simulink model "FS_PWT_Full_Assembly"  (R2025b)
settings: Solver=ode1  StartTime=0.0  StopTime=17  FixedStep=0.05*1/f_sw  RelTol=1e-3
values from neighbouring files (symbols this model uses):
  f_sw = 10000    [Example_parameters.m]
  G_off = 1e-6    (= 1e-06)    [Example_parameters.m]
  J_m = 2.74e-4    (= 0.000274)    [Example_parameters.m]
  k_T = 0.208    [Example_parameters.m]
  n_max = 20000    [Example_parameters.m]
  nm_ref = n_max    (= 20000)    [Example_parameters.m]
  p = 5    [Example_parameters.m]
  R_ds = 0.01    [Example_parameters.m]
  t0 = 0.2    [Example_parameters.m]
  T1 = 0.9*T_max    (= 18)    [Example_parameters.m]
  t1 = t0+5    (= 5.2)    [Example_parameters.m]
  T2 = -T_rated    (= -9.8)    [Example_parameters.m]
  t2 = t1+10    (= 15.2)    [Example_parameters.m]
  Torque_set_matrix = [379.08 379.13 379.18 379.23 379.28 379.33 379.38 379.43 379.48 379.53 379.58 379.63 ... (678 elements, 339x2)]    [Example_torque_reference.mat]
  V_dc = 600    [Example_parameters.m]
  V_th = 2    [Example_parameters.m]
libraries: nesl_utility x15, ee_lib x11, fl_lib x9, eeTransforms x3, simulink x1
settings Model: SimulationMode=accelerator  Creator=giuli  LastModifiedBy=test

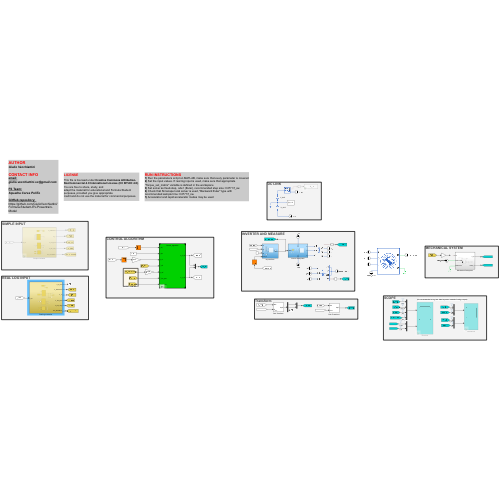
[thumbnail: Simulink's stored preview of the top-level diagram]
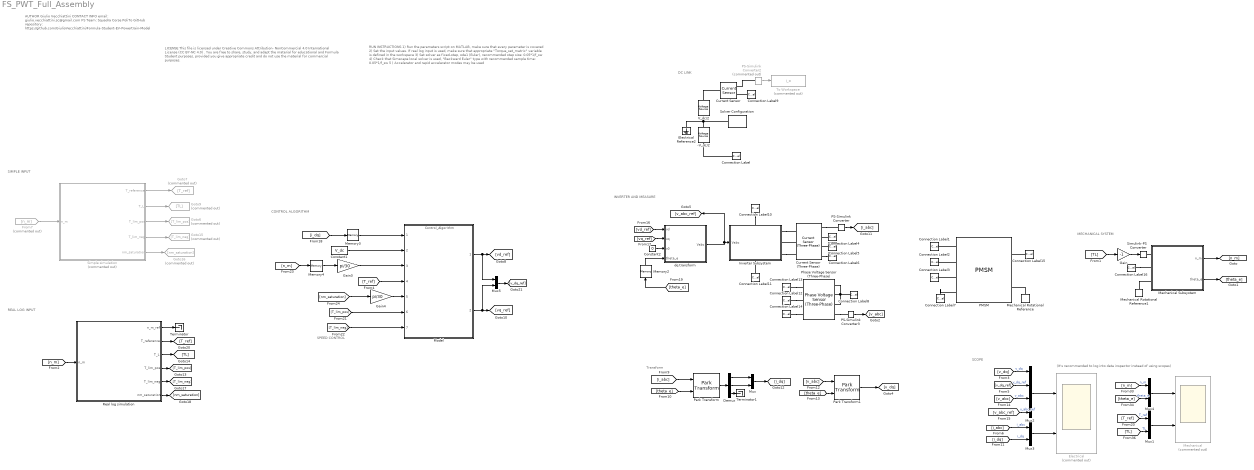
== system FS_PWT_Full_Assembly ==
  note: LICENSE
      |
      | This file is licensed under Creative Commons Attribution-
      | NonCommercial 4.0 International License (CC BY-NC 4.0) . You are free to share, study, and
      | adapt the material for educational and Formula Student purposes, provided you give appropriate
      | credit and do not use the material for commercial purposes.
  note: REAL LOG INPUT
  note: SCOPE
  note: INVERTER AND MEASURE
  note: RUN INSTRUCTIONS
      | 1) Run the parameters script on MATLAB, make sure that every parameter is covered
      | 2) Set the input values. If real log input is used, make sure that appropriate "Torque_set_matrix" variable is defined in the workspace
      | 3) Set solver as fixed-step, ode1 (Euler), recommended step size: 0.05*1/f_sw
      | 4) Check that Simscape local solver is used, "Backward Euler" type with recommended sample time: 0.05*1/f_sw
      | 5 ) Accelerator and rapid accelerator modes may be used
  note: SIMPLE INPUT
  note: DC LINK
  note: Transform
  note: SPEED CONTROL
  note: MECHANICAL SYSTEM
  note: CONTROL ALGORITHM
  note: AUTHOR
      | Giulio Vecchiattini
      |
      | CONTACT INFO
      | email: giulio.vecchiattini.sc@gmail.com
      |
      | FS Team:
      | Squadra Corse PoliTo
      |
      | GitHub repository:
      | https://github.com/GiulioVecchiattini/Formula-Student-EV-Powertrain-Model
  note: (It's recommended to log into data inspector instead of using scopes)
  -V_dc/2 : ee_lib/Sources/Voltage Source  dc_voltage=V_dc/2 V  ac_voltage=0 V  ac_shift=0 rad  ac_frequency=0 Hz  noise_mode=ee.enum.sources.noise.Disabled  PSD=0 V^2/Hz  sample_time=1e-3 s  repeatability=ee.enum.sources.repeatability.NotRepeatable  user_seed=0  auto_seed=2715962282  i_specify=off  i_priority=None  i=0 A  i_nominal_specify=off  i_nominal_value=1  i_nominal_unit=A  v_specify=off  v_priority=None  v=0 V  v_nominal_specify=off  v_nominal_value=1  v_nominal_unit=V
  Connection Label : ConnectionLabel  Label=Neg
  Connection Label1 : ConnectionLabel  Label=v_a
  Connection Label10 : ConnectionLabel  Label=V_dc
  Connection Label11 : ConnectionLabel  Label=Neg
  Connection Label12 : ConnectionLabel  Label=v_b
  Connection Label13 : ConnectionLabel  Label=v_c
  Connection Label14 : ConnectionLabel  Label=v_a
  Connection Label15 : ConnectionLabel  Label=Rotor_shaft
  Connection Label16 : ConnectionLabel  Label=Rotor_shaft
  Connection Label2 : ConnectionLabel  Label=v_b
  Connection Label3 : ConnectionLabel  Label=v_c
  Connection Label4 : ConnectionLabel  Label=v_a
  Connection Label5 : ConnectionLabel  Label=v_b
  Connection Label6 : ConnectionLabel  Label=v_c
  Connection Label7 : ConnectionLabel  Label=motor_ground
  Connection Label8 : ConnectionLabel  Label=motor_ground
  Connection Label9 : ConnectionLabel  Label=V_dc
  Constant1 : Constant  Value=V_dc
  Constant2 : Constant  Value=0
  Current Sensor : fl_lib/Electrical/Electrical Sensors/Current Sensor
  Current Sensor (Three-Phase) : ee_lib/Sensors & Transducers/Current Sensor (Three-Phase)
      settings: InternalSimscapePortConfiguration="{\"Bottom\":[],\"Left\":[{\"id\":\"a1\",\"label\":\"a1\",\"type\":\"foundation.electrical.electrical\"},{\"id\":\"b1\",\"label\":\"b1\",\"type\":\"foundation.electrical.electrical\"},{\"id\":\"c1\",\"label\":\"c1\",\"type\":\"foundation.electrical.electrical\"}],\"Right\":[{\"id\":\"I_output\",\"label\":\"I\",\"type\":\"output\"},{\"id\":\"a2\",\"label\":\"a2\",\"type\":\"foundation.electrical.electrical\"},{\"id\":\"b2\",\"label\":\"b2\",\"type\":\"foundation.electrical.electrical\"},{\"id\":\"c2\",\"label\":\"c2\",\"type\":\"foundation.electrical.electrical\"}],\"Top\":[]}"
  Demux : Demux  Outputs=3
  Electrical : Scope  Commented=on  NumInputPorts=2
      settings: ActiveDisplayYMinimum=-254.85497098950052  ActiveDisplayYMaximum=280.09054138194477
  Electrical Reference2 : fl_lib/Electrical/Electrical Elements/Electrical Reference
  From7 : From  Commented=on  GotoTag=n_m
  Gain : Gain  Gain=-1
  Gain3 : Gain  Gain=pi/30
  Gain4 : Gain  Gain=pi/30
  Goto15 : Goto  Commented=on  GotoTag=T_lim_neg
  Goto16 : Goto  Commented=on  GotoTag=nm_saturation
  Goto6 : Goto  Commented=on  GotoTag=T_lim_pos
  Goto7 : Goto  Commented=on  GotoTag=T_ref
  Goto9 : Goto  Commented=on  GotoTag=TL
  Inverter Subsystem : Subsystem
      settings: PortSchema="{\"entries\":[{\"content\":{\"sides\":[{\"content\":{\"connectorIds\":[\"In1\"]},\"type\":\"ConnectorPlacement.EquallySpacedRectSide\",\"uuid\":\"d192f5af-ddff-4fda-a54c-c11e3916a7bb\"},{\"content\":{\"connectorIds\":[\"RConn1\",\"RConn2\",\"RConn3\"],\"side\":\"RIGHT\"},\"type\":\"ConnectorPlacement.EquallySpacedRectSide\",\"uuid\":\"2c430e4a-8be9-4c5f-98fc-1673ba6cdbf8\"},{\"content\":{\"connectorIds\":[\"LConn1\"],\"side\":\"TOP\"},\"type\":\"ConnectorPlacement.EquallySpacedRectSide\",\"uuid\":\"e498738c-bc20-41e6-88d8-a49171ce1bf1\"},{\"content\":{\"connectorIds\":[\"RConn4\"],\"side\":\"BOTTOM\"},\"type\":\"ConnectorPlacement.EquallySpacedRectSide\",\"uuid\":\"b8f4106f-31ca-4add-9d4b-ac081118ee10\"}]},\"type\":\"ConnectorPlacement.EquallySpacedConnector\",\"uuid\":\"9fb2183f-2e1f-4b7b-94f3-85e82ac3160c\"}],\"packageUris\":[\"http://schema.mathworks.com/mf0/Connector/R2020b\"],\"version\":\"1.0\"}"
  Mechanical : Scope  Commented=on  NumInputPorts=2
      settings: ActiveDisplayYMinimum=-2480.3611684593266  ActiveDisplayYMaximum=22322.963570599019  DataLoggingVariableName=ScopeData5
  Mechanical Rotational Reference : fl_lib/Mechanical/Rotational Elements/Mechanical Rotational Reference
  Mechanical Rotational Reference1 : fl_lib/Mechanical/Rotational Elements/Mechanical Rotational Reference
  Mechanical Subsystem : Subsystem
  Memory2 : Memory
  Memory3 : Memory
  Memory4 : Memory
  Model : ModelReference  ModelNameDialog=Control_Algorithm.slxp  UsingDefaultArgumentValue=0,0,0,0,0,0,0,0,0,0,0,0,0,0,0,0,0,0,0  ModelReferenceVersion=1.7  CopyOfModelProtected=on  Torque_control=0  T_max=T_max  V_dc_max=V_dc_max  V_max=V_max  k_T=k_T  I_max=I_max  Kp_d=Kp_d  Ki_d=Ki_d  Kp_q=Kp_q  Ki_q=Ki_q  Kp_n=Kp_n  Ki_n=Ki_n  Kd_n=Kd_n  Kp_v=Kp_v  Ki_v=Ki_v  n_lim_brake=0.02*n_max  n_min_brake=0.01*n_max  n_max=n_max*1.02  n_lim=0.95*n_max
  Mux{,1,3..5} (5 alike) : Mux  Inputs=2
  Mux2 : Mux
  PMSM : ee_lib/Electromechanical/Permanent Magnet/PMSM  port_option=ee.enum.threePhasePort.expanded  winding_type=ee.enum.electromech.statorconfiguration.wye  machine_param=ee.enum.pmsm.parameterization.constant  nPolePairs=p  pmflux_param=ee.enum.pmflux.fluxlinkage  pm_flux_linkage=Fm Wb  torque_constant=k_T*0.8 N*m/A  back_emf_constant=0.18 V*s/rad  stator_param=ee.enum.statorparam.LdLqL0  Ld=Ld H  Lq=Lq H  idVec=[-200, 0, 200] A  iqVec=[-200, 0, 200] A  LdMatrix=0.0002 * ones(3, 3) H  LqMatrix=0.0002 * ones(3, 3) H  PmMatrix=0.1 * ones(3, 3) Wb  ktMatrix=0.18 * ones(3, 3) N*m/A  keMatrix=0.18 * ones(3, 3) V*s/rad  L0=L0 H  Ls=0.0002 H  Lm=-0.00002 H  Ms=0.00002 H  Rs=R_s Ohm  zero_sequence=ee.enum.park.zerosequence.include  axes_param=ee.enum.rotorangle.daxis  loss_param=ee.enum.ironloss.none  losses_oc=[0, 0, 0] W  losses_sc=[0, 0, 0] W  f_losses=60 Hz  Isc_losses=95 A  J=J_m kg*m^2  lam=B_m N*m*s/rad  i_d_specify=off  i_d_priority=None  i_d=0 A  i_d_nominal_specify=off  i_d_nominal_value=1  i_d_nominal_unit=A  i_q_specify=off  i_q_priority=None  i_q=0 A  i_q_nominal_specify=off  i_q_nominal_value=1  i_q_nominal_unit=A  torque_specify=off  torque_priority=None  torque=0 N*m  torque_nominal_specify=off  torque_nominal_value=1  torque_nominal_unit=N*m  angular_velocity_specify=off  angular_velocity_priority=High  angular_velocity=0 rpm  angular_velocity_nominal_specify=off  angular_velocity_nominal_value=1  angular_velocity_nominal_unit=rpm  angular_position_specify=off  angular_position_priority=High  angular_position=0 deg  angular_position_nominal_specify=off  angular_position_nominal_value=1  angular_position_nominal_unit=deg  alpha=3.93e-3 1/K  alpha_flux=-0.001 1/K  Tmeas=298.15 K  stator_thermal_mass=100 J/K  rotor_thermal_mass=200 J/K  Rm_percent_rotor=90  Rd_percent_rotor=30  temperatureA_specify=off  temperatureA_priority=High  temperatureA=25 degC  temperatureA_nominal_specify=off  temperatureA_nominal_value=1  temperatureA_nominal_unit=degC  temperatureB_specify=off  temperatureB_priority=High  temperatureB=25 degC  temperatureB_nominal_specify=off  temperatureB_nominal_value=1  temperatureB_nominal_unit=degC  temperatureC_specify=off  temperatureC_priority=High  temperatureC=25 degC  temperatureC_nominal_specify=off  temperatureC_nominal_value=1  temperatureC_nominal_unit=degC  temperatureR_specify=off  temperatureR_priority=High  temperatureR=25 degC  temperatureR_nominal_specify=off  temperatureR_nominal_value=1  temperatureR_nominal_unit=degC
      settings: InternalSimscapePortConfiguration="{\"Bottom\":[],\"Left\":[{\"id\":\"a\",\"label\":\"a\",\"type\":\"foundation.electrical.electrical\"},{\"id\":\"b\",\"label\":\"b\",\"type\":\"foundation.electrical.electrical\"},{\"id\":\"c\",\"label\":\"c\",\"type\":\"foundation.electrical.electrical\"},{\"id\":\"n\",\"label\":\"n\",\"type\":\"foundation.electrical.electrical\"}],\"Right\":[{\"id\":\"R\",\"label\":\"R\",\"type\":\"foundation.mechanical.rotational.rotational\"},{\"id\":\"C\",\"label\":\"C\",\"type\":\"foundation.mechanical.rotational.rotational\"}],\"Top\":[]}"
  PS-Simulink Converter : nesl_utility/PS-Simulink Converter  PhysicalDomain=network_engine_domain  SubClassName=ps_output  LeftPortType=input  RightPortType=output  PseudoPeriodic=off  Frequencies=[]  VectorFormat=inherit  Unit=inherit  AffineConversion=off
  PS-Simulink Converter2 : nesl_utility/PS-Simulink Converter  Commented=on  PhysicalDomain=network_engine_domain  SubClassName=ps_output  LeftPortType=input  RightPortType=output  PseudoPeriodic=off  Frequencies=[]  VectorFormat=inherit  Unit=inherit  AffineConversion=off
  PS-Simulink Converter3 : nesl_utility/PS-Simulink Converter  PhysicalDomain=network_engine_domain  SubClassName=ps_output  LeftPortType=input  RightPortType=output  PseudoPeriodic=off  Frequencies=[]  VectorFormat=inherit  Unit=inherit  AffineConversion=off
  Park Transform : eeTransforms/Park Transform  AxisAlignment=D-axis  PowerInvariant=off
      settings: LibrarySourceBlock=|
      | ee_sl_lib/Mathematical
      | Transforms/Park Transform
  Park Transform1 : eeTransforms/Park Transform  AxisAlignment=D-axis  PowerInvariant=off
      settings: LibrarySourceBlock=|
      | ee_sl_lib/Mathematical
      | Transforms/Park Transform
  Phase Voltage Sensor (Three-Phase) : ee_lib/Sensors & Transducers/Phase Voltage Sensor (Three-Phase)
      settings: InternalSimscapePortConfiguration="{\"Bottom\":[],\"Left\":[{\"id\":\"a1\",\"label\":\"a1\",\"type\":\"foundation.electrical.electrical\"},{\"id\":\"b1\",\"label\":\"b1\",\"type\":\"foundation.electrical.electrical\"},{\"id\":\"c1\",\"label\":\"c1\",\"type\":\"foundation.electrical.electrical\"}],\"Right\":[{\"id\":\"V_output\",\"label\":\"V\",\"type\":\"output\"},{\"id\":\"a2\",\"label\":\"a2\",\"type\":\"foundation.electrical.electrical\"},{\"id\":\"b2\",\"label\":\"b2\",\"type\":\"foundation.electrical.electrical\"},{\"id\":\"c2\",\"label\":\"c2\",\"type\":\"foundation.electrical.electrical\"}],\"Top\":[]}"
  Real log simulation : Subsystem
  Simple simulation : Subsystem  Commented=on
  Simulink-PS Converter : nesl_utility/Simulink-PS Converter  PhysicalDomain=network_engine_domain  SubClassName=ps_input  LeftPortType=input  RightPortType=output  PseudoPeriodic=off  Frequencies=[]  NoiseDistribution=none  NoiseParameters=[]  Unit=1  AffineConversion=off  FilteringAndDerivatives=provide  SimscapeFilterOrder=1  InputFilterTimeConstant=0.001  UdotUserProvided=0
  Solver Configuration : nesl_utility/Solver Configuration  PhysicalDomain=network_engine_domain  SubClassName=solver  LeftPortType=input  RightPortType=generic  Tones=[]  Harmonics=[]  SimulateNoise=off  Profile=off  UseLocalSampling=off  EnableSwitchedLinearOptims=on  FrequencyDomain=off  UseCCode=off  RelTol=0.001  AbsTol=0.001  MinStep=1e-09  ToWorkspace=off  RevertToSquareIcSolve=off  NumHomotopyIterations=100  PhasorMode=off  PhasorModeNumHarmonics=1  ConsistencySolver=NEWTON_XTOL_AFTER_FTOL  IndexReductionMethod=DerivativeReplacement  DoDC=off  ResidualTolerance=1e-09  ConsistencyTolSource=GLOBAL  ConsistencyAbsTol=0.001  ConsistencyRelTol=0.001  ConsistencyTolFactor=0.001  UseLocalSolver=on  LocalSolverChoice=NE_BACKWARD_EULER_ADVANCER  ResolveIndetEquations=on  FunctionEvalNumThread=1  LocalSolverSampleTime=0.5*0.1*1/f_sw  DoFixedCost=off  MaxNonlinIter=3  MaxModeIter=2  ComputeImpulses=off  ImpulseIterations=2  LinearAlgebra=auto  LinearAlgebraNumThread=0  EquationFormulation=NE_TIME_EF  DelaysMemoryBudget=1024  AutomaticFiltering=on  FilteringTimeConstant=0.001  PartitionStorageMethod=AS_NEEDED  PartitionMemoryBudget=1024  PartitionMethod=ROBUST  MultibodyUseLocalSolver=off  MultibodyLocalSolverChoice=ODE1  MultibodyLocalSolverSampleTime=0.001
  Terminator : Terminator
  Terminator1 : Terminator
  To Workspace : ToWorkspace  Commented=on  VariableName=i_o  SampleTime=-1
      settings: Save2DSignal=2-D array (concatenate along first dimension)
  V_dc/2 : ee_lib/Sources/Voltage Source  dc_voltage=V_dc/2 V  ac_voltage=0 V  ac_shift=0 rad  ac_frequency=0 Hz  noise_mode=ee.enum.sources.noise.Disabled  PSD=0 V^2/Hz  sample_time=1e-3 s  repeatability=ee.enum.sources.repeatability.NotRepeatable  user_seed=0  auto_seed=418932850  i_specify=off  i_priority=None  i=0 A  i_nominal_specify=off  i_nominal_value=1  i_nominal_unit=A  v_specify=off  v_priority=None  v=0 V  v_nominal_specify=off  v_nominal_value=1  v_nominal_unit=V
  dq transform : Subsystem
  wires:
  [n_m] -> Real log simulation/1(n_m)
  Real log simulation/1(n_m_ref) -> Terminator/1
  [vd_ref] -> dq transform/1(vd)
  [n_m] -> Mux4/1  "n_m"
  Simple simulation/2(T_L) -> Goto9/1
  PS-Simulink Converter2/1 -> To Workspace/1
  [T_ref] -> Model/4
  Gain/1 -> Simulink-PS Converter/1
  [v_dq_ref] -> Mux2/2  "v_dq_ref"
  [theta_e] -> Park Transform1/2
  Model/1 -> Mux5/1, [vd_ref]
  [n_m] -> Memory4/1
  Memory3/1 -> Model/1
  Real log simulation/3(T_L) -> [TL]
  Mux3/1 -> Electrical/2
  Mechanical Subsystem/1(n_m) -> [n_m]
  [T_ref] -> Mux1/1  "T_ref"
  [T_lim_pos] -> Model/6
  [i_dq] -> Memory3/1
  [i_dq] -> Mux3/2  "i_dq"
  [i_abc] -> Mux3/1  "i_abc"
  Real log simulation/5(T_lim_neg) -> [T_lim_neg]
  Park Transform1/1 -> [v_dq]
  Real log simulation/4(T_lim_pos) -> [T_lim_pos]
  [v_dq] -> Mux2/1  "v_dq"
  [vq_ref] -> dq transform/2(vq)
  [theta_e] -> Park Transform/2
  Mux5/1 -> [v_dq_ref]
  PS-Simulink Converter3/1 -> [v_abc]
  Mechanical Subsystem/2(theta_e) -> [theta_e]
  Memory4/1 -> Gain3/1
  Constant1/1 -> Model/2
  [v_abc_ref] -> Mux2/4  "v_abc_ref"
  [TL] -> Gain/1
  Gain3/1 -> Model/3
  Mux1/1 -> Mechanical/2
  Real log simulation/2(T_reference) -> [T_ref]
  Real log simulation/6(nm_saturation) -> [nm_saturation]
  Mux4/1 -> Mechanical/1
  [TL] -> Mux1/2  "TL"
  Constant2/1 -> dq transform/3(v0)
  [v_abc] -> Mux2/3  "v_abc"
  PS-Simulink Converter/1 -> [i_abc]
  dq transform/1(Vabc) -> [v_abc_ref], Inverter Subsystem/1(Vabc)
  Mux2/1 -> Electrical/1
  [i_abc] -> Park Transform/1
  Model/2 -> Mux5/2, [vq_ref]
  Simple simulation/1(T_reference) -> Goto7/1
  [nm_saturation] -> Gain4/1
  [theta_e] -> Mux4/2  "theta_e"
  [v_abc] -> Park Transform1/1
  [theta_e] -> Memory2/1
  [T_lim_neg] -> Model/7
  Memory2/1 -> dq transform/4(theta_e)
  Gain4/1 -> Model/5
  Demux/2 -> Mux/2
  Demux/1 -> Mux/1
  Demux/3 -> Terminator1/1
  Mux/1 -> [i_dq]
  Park Transform/1 -> Demux/1
  From7/1 -> Simple simulation/1(n_m)
  Simple simulation/3(T_lim_pos) -> Goto6/1
  Simple simulation/4(T_lim_neg) -> Goto15/1
  Simple simulation/5(nm_saturation) -> Goto16/1
  connections:
  Phase Voltage Sensor (Three-Phase)/RConn3 -- Phase Voltage Sensor (Three-Phase)/RConn2 -- Phase Voltage Sensor (Three-Phase)/RConn4 -- Connection Label8/LConn1
  V_dc/2/RConn1 -- -V_dc/2/LConn1 -- Solver Configuration/RConn1 -- Electrical Reference2/LConn1
  Current Sensor/RConn1 -- PS-Simulink Converter2/LConn1
  Connection Label/LConn1 -- -V_dc/2/RConn1
  Inverter Subsystem/RConn1 -- Current Sensor (Three-Phase)/LConn1
  Connection Label16/LConn1 -- Mechanical Subsystem/LConn2
  Current Sensor (Three-Phase)/LConn2 -- Inverter Subsystem/RConn2
  Current Sensor (Three-Phase)/RConn1 -- PS-Simulink Converter/LConn1
  Phase Voltage Sensor (Three-Phase)/RConn1 -- PS-Simulink Converter3/LConn1
  Connection Label12/LConn1 -- Phase Voltage Sensor (Three-Phase)/LConn2
  Mechanical Rotational Reference/LConn1 -- PMSM/RConn2
  Connection Label11/LConn1 -- Inverter Subsystem/RConn4
  PMSM/LConn1 -- Connection Label1/LConn1
  Simulink-PS Converter/RConn1 -- Mechanical Subsystem/LConn1
  Connection Label15/LConn1 -- PMSM/RConn1
  Connection Label7/LConn1 -- PMSM/LConn4
  PMSM/LConn3 -- Connection Label3/LConn1
  Mechanical Rotational Reference1/LConn1 -- Mechanical Subsystem/LConn3
  Connection Label14/LConn1 -- Phase Voltage Sensor (Three-Phase)/LConn1
  PMSM/LConn2 -- Connection Label2/LConn1
  Connection Label4/LConn1 -- Current Sensor (Three-Phase)/RConn2
  Connection Label9/LConn1 -- Current Sensor/RConn2
  V_dc/2/LConn1 -- Current Sensor/LConn1
  Connection Label10/LConn1 -- Inverter Subsystem/LConn1
  Connection Label13/LConn1 -- Phase Voltage Sensor (Three-Phase)/LConn3
  Inverter Subsystem/RConn3 -- Current Sensor (Three-Phase)/LConn3
  Current Sensor (Three-Phase)/RConn4 -- Connection Label6/LConn1
  Connection Label5/LConn1 -- Current Sensor (Three-Phase)/RConn3

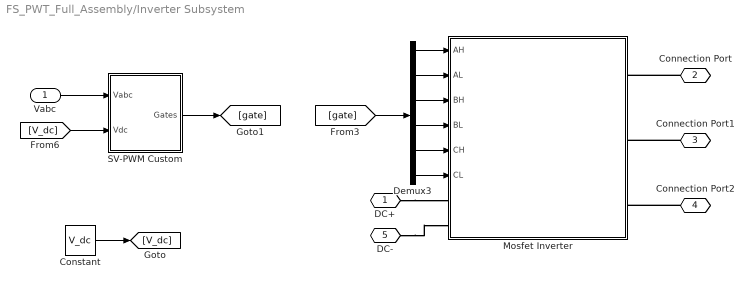
== system FS_PWT_Full_Assembly/Inverter Subsystem ==
  Vabc : Inport
  Constant : Constant  Value=V_dc
  Demux3 : Demux  Outputs=6
  Mosfet Inverter : Subsystem  mask(Custom Inverter){R_DS=R_ds, G_off=G_off, V_th=V_th}
      mask prompts: R_DS "Drain-source resistance (Ohm)"; G_off "Off conductance (1/Ohm)"; V_th "Treshold voltage"
      mask help: Custom mosfet inverter
      mask DialogControl ParameterGroupVar Prompt: MOSFET parameters
      mask Display: image('Inverter_mask.png');
  SV-PWM Custom : Subsystem  mask(Space Vector PWM Modulator){f_sw=f_sw, G_pulse=10}
      mask prompts: f_sw "Switching frequency (Hz)"; G_pulse "Gate pulse amplitude (V)"
      mask help: SV-PWM Modulator with common mode modulation injection, triangular carrier based
  DC+ : PMIOPort  Side=Left
  Connection Port : PMIOPort  Port=2  Side=Right
  Connection Port1 : PMIOPort  Port=3  Side=Right
  Connection Port2 : PMIOPort  Port=4  Side=Right
  DC- : PMIOPort  Port=5  Side=Right
  wires:
  [V_dc] -> SV-PWM Custom/2(Vdc)
  Demux3/4 -> Mosfet Inverter/4(BL)
  Demux3/2 -> Mosfet Inverter/2(AL)
  Demux3/6 -> Mosfet Inverter/6(CL)
  [gate] -> Demux3/1
  Demux3/3 -> Mosfet Inverter/3(BH)
  Demux3/1 -> Mosfet Inverter/1(AH)
  Demux3/5 -> Mosfet Inverter/5(CH)
  SV-PWM Custom/1(Gates) -> [gate]
  Vabc/1 -> SV-PWM Custom/1(Vabc)
  Constant/1 -> [V_dc]
  connections:
  DC+/RConn1 -- Mosfet Inverter/LConn1
  DC-/RConn1 -- Mosfet Inverter/LConn2
  Connection Port/RConn1 -- Mosfet Inverter/RConn1
  Connection Port1/RConn1 -- Mosfet Inverter/RConn2
  Connection Port2/RConn1 -- Mosfet Inverter/RConn3

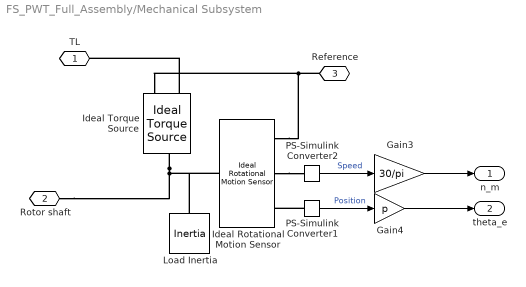
== system FS_PWT_Full_Assembly/Mechanical Subsystem ==
  Gain3 : Gain  Gain=30/pi
  Gain4 : Gain  Gain=p
  Ideal Rotational Motion Sensor : fl_lib/Mechanical/Mechanical Sensors/Ideal Rotational Motion Sensor  reference=foundation.enum.MeasurementReference.difference  acceleration_port=false  velocity_port=true  position_port=true  wrap_angle=true  offset=0 rad
  Ideal Torque Source : fl_lib/Mechanical/Mechanical Sources/Ideal Torque Source
  Load Inertia : fl_lib/Mechanical/Rotational Elements/Inertia  inertia=J_eq kg*m^2  num_ports=foundation.enum.numPorts2.one  w_specify=off  w_priority=High  w=0 rad/s  w_nominal_specify=off  w_nominal_value=1  w_nominal_unit=rad/s  t_specify=off  t_priority=None  t=0 N*m  t_nominal_specify=off  t_nominal_value=1  t_nominal_unit=N*m
  PS-Simulink Converter1 : nesl_utility/PS-Simulink Converter  PhysicalDomain=network_engine_domain  SubClassName=ps_output  LeftPortType=input  RightPortType=output  PseudoPeriodic=off  Frequencies=[]  VectorFormat=inherit  Unit=inherit  AffineConversion=off
  PS-Simulink Converter2 : nesl_utility/PS-Simulink Converter  PhysicalDomain=network_engine_domain  SubClassName=ps_output  LeftPortType=input  RightPortType=output  PseudoPeriodic=off  Frequencies=[]  VectorFormat=inherit  Unit=inherit  AffineConversion=off
  TL : PMIOPort  Side=Left
  Rotor shaft : PMIOPort  Port=2  Side=Left
  Reference : PMIOPort  Port=3  Side=Left
  n_m : Outport
  theta_e : Outport  Port=2
  wires:
  PS-Simulink Converter2/1 -> Gain3/1  "Speed"
  PS-Simulink Converter1/1 -> Gain4/1  "Position"
  Gain4/1 -> theta_e/1
  Gain3/1 -> n_m/1
  connections:
  Ideal Torque Source/LConn1 -- Rotor shaft/RConn1 -- Ideal Rotational Motion Sensor/LConn1 -- Load Inertia/LConn1
  Ideal Torque Source/RConn1 -- TL/RConn1
  PS-Simulink Converter1/LConn1 -- Ideal Rotational Motion Sensor/RConn3
  Ideal Rotational Motion Sensor/RConn1 -- Reference/RConn1 -- Ideal Torque Source/RConn2
  Ideal Rotational Motion Sensor/RConn2 -- PS-Simulink Converter2/LConn1

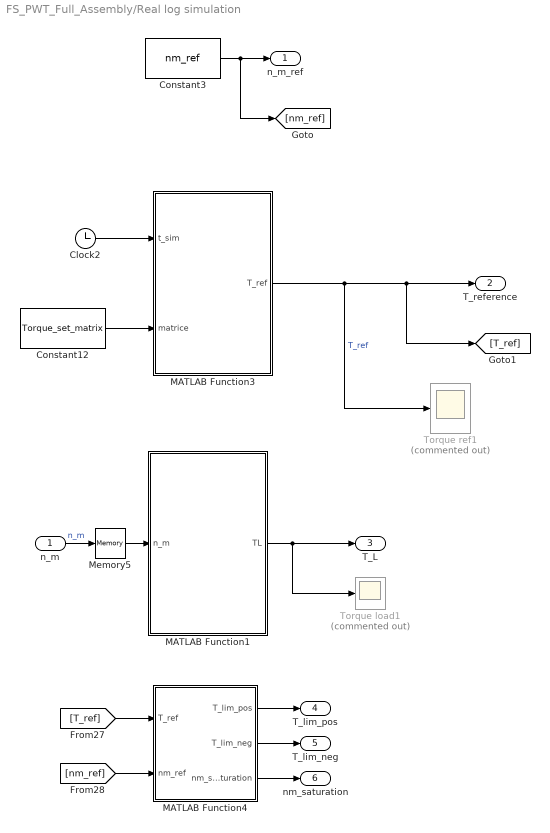
== system FS_PWT_Full_Assembly/Real log simulation ==
  n_m : Inport
  Clock2 : Clock
  Constant12 : Constant  Value=Torque_set_matrix
  Constant3 : Constant  Value=nm_ref
  MATLAB Function1 : MATLAB Function  TreatAsAtomicUnit=on
  MATLAB Function3 : MATLAB Function  TreatAsAtomicUnit=on
  MATLAB Function4 : MATLAB Function  TreatAsAtomicUnit=on
  Memory5 : Memory
  Torque load1 : Scope  Commented=on
      settings: ActiveDisplayYMinimum=-0.11038663411275673  ActiveDisplayYMaximum=2.0946275210188139
  Torque ref1 : Scope  Commented=on
      settings: ActiveDisplayYMinimum=-0.84016888799599976  ActiveDisplayYMaximum=7.5615199919639995  DataLoggingVariableName=ScopeData2
  n_m_ref : Outport
  T_reference : Outport  Port=2
  T_L : Outport  Port=3
  T_lim_pos : Outport  Port=4
  T_lim_neg : Outport  Port=5
  nm_saturation : Outport  Port=6
  wires:
  MATLAB Function4/1(T_lim_pos) -> T_lim_pos/1
  MATLAB Function4/3(nm_saturation) -> nm_saturation/1
  MATLAB Function1/1(TL) -> T_L/1, Torque load1/1
  n_m/1 -> Memory5/1  "n_m"
  MATLAB Function4/2(T_lim_neg) -> T_lim_neg/1
  [nm_ref] -> MATLAB Function4/2(nm_ref)
  [T_ref] -> MATLAB Function4/1(T_ref)
  Constant12/1 -> MATLAB Function3/2(matrice)
  Memory5/1 -> MATLAB Function1/1(n_m)
  Clock2/1 -> MATLAB Function3/1(t_sim)
  MATLAB Function3/1(T_ref) -> [T_ref], T_reference/1, Torque ref1/1  "T_ref"
  Constant3/1 -> [nm_ref], n_m_ref/1

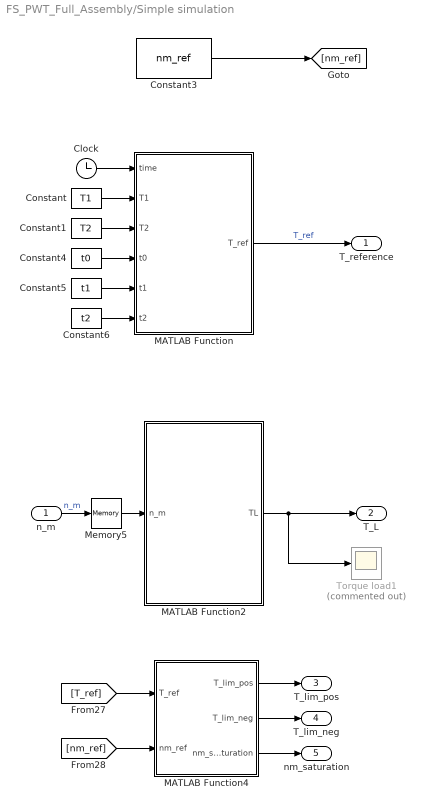
== system FS_PWT_Full_Assembly/Simple simulation ==
  n_m : Inport
  Clock : Clock
  Constant : Constant  Value=T1
  Constant1 : Constant  Value=T2
  Constant3 : Constant  Value=nm_ref
  Constant4 : Constant  Value=t0
  Constant5 : Constant  Value=t1
  Constant6 : Constant  Value=t2
  MATLAB Function : MATLAB Function  TreatAsAtomicUnit=on
  MATLAB Function2 : MATLAB Function  TreatAsAtomicUnit=on
  MATLAB Function4 : MATLAB Function  TreatAsAtomicUnit=on
  Memory5 : Memory
  Torque load1 : Scope  Commented=on
      settings: ActiveDisplayYMinimum=-0.11038663411275673  ActiveDisplayYMaximum=2.0946275210188139  DataLoggingVariableName=ScopeData3
  T_reference : Outport
  T_L : Outport  Port=2
  T_lim_pos : Outport  Port=3
  T_lim_neg : Outport  Port=4
  nm_saturation : Outport  Port=5
  wires:
  Constant/1 -> MATLAB Function/2(T1)
  Constant6/1 -> MATLAB Function/6(t2)
  Clock/1 -> MATLAB Function/1(time)
  Constant4/1 -> MATLAB Function/4(t0)
  Constant1/1 -> MATLAB Function/3(T2)
  Constant5/1 -> MATLAB Function/5(t1)
  MATLAB Function/1(T_ref) -> T_reference/1  "T_ref"
  Constant3/1 -> [nm_ref]
  n_m/1 -> Memory5/1  "n_m"
  Memory5/1 -> MATLAB Function2/1(n_m)
  MATLAB Function2/1(TL) -> T_L/1, Torque load1/1
  MATLAB Function4/1(T_lim_pos) -> T_lim_pos/1
  MATLAB Function4/2(T_lim_neg) -> T_lim_neg/1
  [nm_ref] -> MATLAB Function4/2(nm_ref)
  [T_ref] -> MATLAB Function4/1(T_ref)
  MATLAB Function4/3(nm_saturation) -> nm_saturation/1

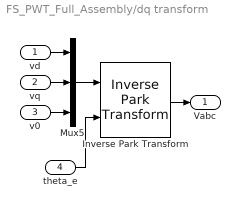
== system FS_PWT_Full_Assembly/dq transform ==
  vd : Inport
  vq : Inport  Port=2
  v0 : Inport  Port=3
  theta_e : Inport  Port=4
  Inverse Park Transform : eeTransforms/Inverse Park Transform  AxisAlignment=D-axis  PowerInvariant=off
      settings: LibrarySourceBlock=|
      | ee_sl_lib/Mathematical
      | Transforms/Inverse
      | Park Transform
  Mux5 : Mux  Inputs=3
  Vabc : Outport
  wires:
  vd/1 -> Mux5/1
  Mux5/1 -> Inverse Park Transform/1
  Inverse Park Transform/1 -> Vabc/1
  vq/1 -> Mux5/2
  v0/1 -> Mux5/3
  theta_e/1 -> Inverse Park Transform/2

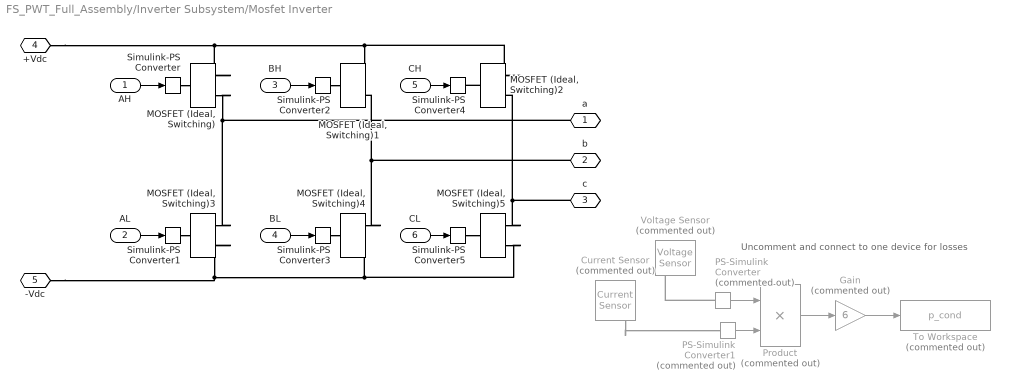
== system FS_PWT_Full_Assembly/Inverter Subsystem/Mosfet Inverter ==
  note: Uncomment and connect to one device for losses
  AH : Inport
  AL : Inport  Port=2
  BH : Inport  Port=3
  BL : Inport  Port=4
  CH : Inport  Port=5
  CL : Inport  Port=6
  Current Sensor : fl_lib/Electrical/Electrical Sensors/Current Sensor  Commented=on
  Gain : Gain  Commented=on  Gain=6
  MOSFET (Ideal, Switching){,1..5} (6 alike) : ee_lib/Semiconductors & Converters/MOSFET (Ideal, Switching)  port_option=ee.enum.controlport.ps  Rds=R_DS Ohm  Goff=G_off 1/Ohm  Vth=V_th V  diode_param=ee.enum.semiconductors.protectionDiode.nodynamics  diode_Vf=0.8 V  diode_Ron=0.001 Ohm  diode_Goff=1e-5 1/Ohm  diode_C=50e-9 F  diode_iRM=-235 A  diode_iF=300 A  diode_idot=-50 A/us  diode_trr_param=ee.enum.converters.diodeReverseParam.trr_factor  diode_trr_factor=3  diode_trr=15 us  diode_Qrr=1500 s*uA  ids_specify=off  ids_priority=None  ids=0 A  ids_nominal_specify=off  ids_nominal_value=1  ids_nominal_unit=A  vds_specify=off  vds_priority=None  vds=0 V  vds_nominal_specify=off  vds_nominal_value=1  vds_nominal_unit=V  vgs_specify=off  vgs_priority=None  vgs=0 V  vgs_nominal_specify=off  vgs_nominal_value=1  vgs_nominal_unit=V  thermal_loss_option=ee.enum.converters.thermalLossOption.constantvalues  Von_data=[0, 1.8, 3.2, 6, 10, 16; 0, 2, 5.5, 9.5, 15, 25] V  Tj=[298.15, 448.15] K  Iout_data=[0, 20, 40, 60, 80, 100] A  Eon_data=[0, 55.04, 124.57, 235.53, 362.12; 0, 71.25, 161.25, 304.88, 468.75] * 1e-6 J  Eoff_data=[0, 18, 30, 56.1, 76.5; 0, 22.5, 37.5, 70.13, 95.63] * 1e-6 J  Eon_data_3D=[zeros(2, 5, 3)] J  Eoff_data_3D=[zeros(2, 5, 3)] J  Tj_loss=[298.15, 448.15] K  Iout_data_loss=[0, 10, 20, 30, 40] A  tabulateWithVds=false  Vds_loss=[0, 150, 300] V  Eon_scalar=22.86e-3 J  Eoff_scalar=17.14e-3 J  Voff=300 V  Iout_scalar=600 A  useCurrentFromPreviousCycle=false  useVoltageFromPreviousCycle=false  diodeModelType=ee.enum.converters.diodeModelType.pwl  diodeTableType=ee.enum.diode.tableType.IfMat  diode_ReverseIVType=ee.enum.diode.diodeReverseIV.constant  diode_IfMat=[.07, .12, .19, 1.75, 4.24, 7.32, 11.2; .16, .3, .72, 2.14, 4.02, 6.35, 9.12] A  diode_VfMat=[.9, 1.15, 1.25, 1.5, 1.75, 2.17, 2.6, 2.85; .58, .68, .75, 1.1, 1.38, 1.77, 2.27, 2.7] V  diode_TjVec=[25, 125] degC  diode_VfVec=[.5, .7, .9, 1.3, 1.7, 2.1, 2.5] V  diode_IfVec=[.1, .2, .5, 1, 2, 4, 7, 10] A  diode_IrMat=[1e-06, 2e-06, 5e-06, 1e-05, 2.5e-05, 5e-05, .0001; 2e-06, 5e-06, 1e-05, 4e-05, 8e-05, .0002, .0005] A  diode_VrMat=[10, 100, 200, 250, 300, 325, 350; 10, 70, 160, 220, 270, 300, 320] V  diode_VrVec=[10, 20, 40, 50, 70, 80, 100] V  diode_IrVec=[1e-06, 2e-06, 5e-06, 1e-05, 2e-05, 5e-05, .0001] A  diode_Vr=-600 V  diode_Ls=150 nH  diode_Erec=0.03 J  diode_rec_loss_model=ee.enum.diode.reverseRecoveryModel.fixed  diode_ErecVal=0 J  diode_scaleWithIandV=true  diode_ErecMat=zeros(2, 3) J  diode_TjrecVec=[298.15, 398.15] K  diode_IfrecVec=[.1, 1, 10] A  diode_IrecVal=10 A  diode_VrecVal=10 V  diode_tFilter=1 / 1000 / 100 s  separateThermalPortForDiode=false  thermal_network_parameterization=ee.enum.thermalNetworkTopology.external  Rth=[.03, .2] K/W  Rth_Cauer=[.03, .1, .2] K/W  Rth_Foster=[.08, .14, .22, .16] K/W  thermal_mass_parameterization=ee.enum.thermalNetwork.timeconstant  thermal_mass=[3, 25] J/K  thermal_mass_Cauer=[3, 10, 25] J/K  thermal_mass_Foster=[.001, .005, .05, .5] J/K  thermal_time_constant=[.1, 5] s  thermal_time_constant_Cauer=[.1, 1, 5] s  thermal_time_constant_Foster=[7e-05, .0007, .01, .08] s  thermal_mass_initial_temperatures=[25, 25] degC  thermal_mass_initial_temperatures_Cauer=[25, 25, 25] degC  junction_thermal_mass=0.1 J/K  Tvec_initial_Foster=[25, 25, 25, 25] degC  RthDiode=[.03, .2] K/W  RthCauerDiode=[.03, .1, .2] K/W  RthFosterDiode=[.03, .2] K/W  thermalMassDiode=[3, 25] J/K  thermalMassCauerDiode=[3, 10, 25] J/K  thermalMassFosterDiode=[33, 50] J/K  thermalTauDiode=[.1, 5] s  thermalTauCauerDiode=[.1, 1, 5] s  thermalTauFosterDiode=[1, 10] s  thermalMassInitTempDiode=[25, 25] degC  thermalMassInitTempCauerDiode=[25, 25, 25] degC  junctionthermalMassDiode=0.1 J/K  TVecInitialFosterDiode=[25, 25, 25, 25] degC  no_thermal_network=0  mosfet_junction_temperature_specify=off  mosfet_junction_temperature_priority=None  mosfet_junction_temperature=25 degC  mosfet_junction_temperature_nominal_specify=off  mosfet_junction_temperature_nominal_value=1  mosfet_junction_temperature_nominal_unit=degC  diode_junction_temperature_specify=off  diode_junction_temperature_priority=None  diode_junction_temperature=25 degC  diode_junction_temperature_nominal_specify=off  diode_junction_temperature_nominal_value=1  diode_junction_temperature_nominal_unit=degC  Qj_specify=off  Qj_priority=None  Qj=0 W  Qj_nominal_specify=off  Qj_nominal_value=1  Qj_nominal_unit=W  accumulatedSwitchingLosses_specify=off  accumulatedSwitchingLosses_priority=None  accumulatedSwitchingLosses=0 J
  PS-Simulink Converter : nesl_utility/PS-Simulink Converter  Commented=on  PhysicalDomain=network_engine_domain  SubClassName=ps_output  LeftPortType=input  RightPortType=output  PseudoPeriodic=off  Frequencies=[]  VectorFormat=inherit  Unit=inherit  AffineConversion=off
  PS-Simulink Converter1 : nesl_utility/PS-Simulink Converter  Commented=on  PhysicalDomain=network_engine_domain  SubClassName=ps_output  LeftPortType=input  RightPortType=output  PseudoPeriodic=off  Frequencies=[]  VectorFormat=inherit  Unit=inherit  AffineConversion=off
  Product : Product  Commented=on
  Simulink-PS Converter{,1..5} (6 alike) : nesl_utility/Simulink-PS Converter  PhysicalDomain=network_engine_domain  SubClassName=ps_input  LeftPortType=input  RightPortType=output  PseudoPeriodic=off  Frequencies=[]  NoiseDistribution=none  NoiseParameters=[]  Unit=1  AffineConversion=off  FilteringAndDerivatives=provide  SimscapeFilterOrder=1  InputFilterTimeConstant=0.001  UdotUserProvided=0
  To Workspace : ToWorkspace  Commented=on  VariableName=p_cond  SaveFormat=Structure With Time  SampleTime=-1
  Voltage Sensor : fl_lib/Electrical/Electrical Sensors/Voltage Sensor  Commented=on
  a : PMIOPort  Side=Right
  b : PMIOPort  Port=2  Side=Right
  c : PMIOPort  Port=3  Side=Right
  +Vdc : PMIOPort  Port=4  Side=Left
  -Vdc : PMIOPort  Port=5  Side=Left
  wires:
  AH/1 -> Simulink-PS Converter/1
  BH/1 -> Simulink-PS Converter2/1
  BL/1 -> Simulink-PS Converter3/1
  AL/1 -> Simulink-PS Converter1/1
  CH/1 -> Simulink-PS Converter4/1
  CL/1 -> Simulink-PS Converter5/1
  PS-Simulink Converter/1 -> Product/1
  PS-Simulink Converter1/1 -> Product/2
  Product/1 -> Gain/1
  Gain/1 -> To Workspace/1
  connections:
  "MOSFET (Ideal, Switching)4"/RConn1 -- b/RConn1 -- "MOSFET (Ideal, Switching)1"/RConn2
  a/RConn1 -- "MOSFET (Ideal, Switching)"/RConn2 -- "MOSFET (Ideal, Switching)3"/RConn1
  "MOSFET (Ideal, Switching)3"/RConn2 -- -Vdc/RConn1 -- "MOSFET (Ideal, Switching)5"/RConn2 -- "MOSFET (Ideal, Switching)4"/RConn2
  "MOSFET (Ideal, Switching)"/RConn1 -- "MOSFET (Ideal, Switching)2"/RConn1 -- "MOSFET (Ideal, Switching)1"/RConn1 -- +Vdc/RConn1
  "MOSFET (Ideal, Switching)5"/RConn1 -- "MOSFET (Ideal, Switching)2"/RConn2 -- c/RConn1
  Simulink-PS Converter/RConn1 -- "MOSFET (Ideal, Switching)"/LConn1
  Simulink-PS Converter1/RConn1 -- "MOSFET (Ideal, Switching)3"/LConn1
  Simulink-PS Converter2/RConn1 -- "MOSFET (Ideal, Switching)1"/LConn1
  Simulink-PS Converter3/RConn1 -- "MOSFET (Ideal, Switching)4"/LConn1
  Simulink-PS Converter5/RConn1 -- "MOSFET (Ideal, Switching)5"/LConn1
  "MOSFET (Ideal, Switching)2"/LConn1 -- Simulink-PS Converter4/RConn1
  PS-Simulink Converter/LConn1 -- Voltage Sensor/RConn1
  Current Sensor/RConn1 -- PS-Simulink Converter1/LConn1

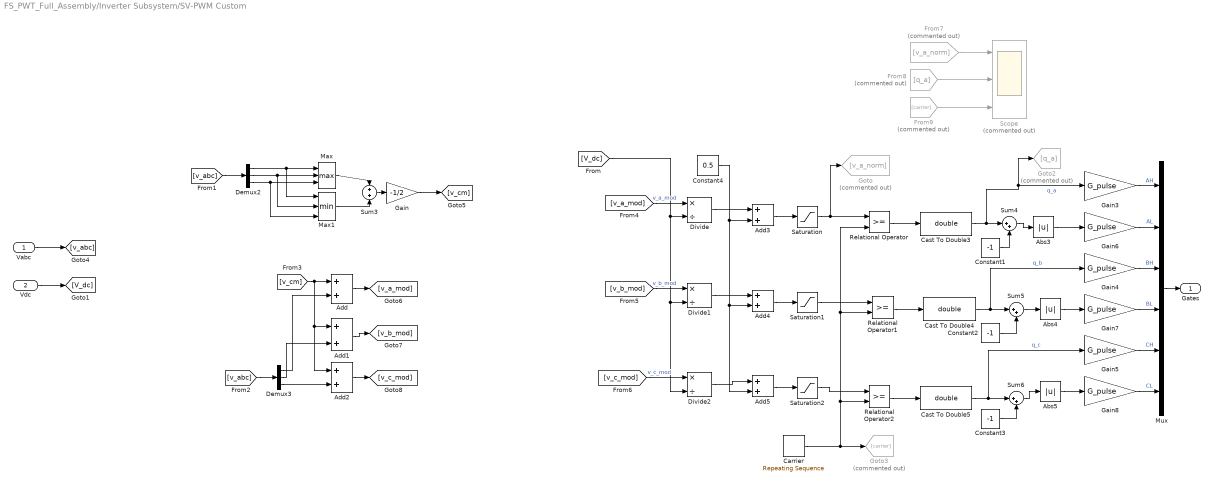
== system FS_PWT_Full_Assembly/Inverter Subsystem/SV-PWM Custom ==
  Vabc : Inport
  Vdc : Inport  Port=2
  Abs3 : Abs  SaturateOnIntegerOverflow=off
  Abs4 : Abs  SaturateOnIntegerOverflow=off
  Abs5 : Abs  SaturateOnIntegerOverflow=off
  Add{,1..5} (6 alike) : Sum
  Carrier : simulink/Sources/Repeating Sequence  rep_seq_t=[0 1/(2*f_sw) 1/f_sw]  rep_seq_y="[0  1 0]"
  Cast To Double3 : DataTypeConversion  OutDataTypeStr=double  SaturateOnIntegerOverflow=off  RndMeth=Floor
  Cast To Double4 : DataTypeConversion  OutDataTypeStr=double  SaturateOnIntegerOverflow=off  RndMeth=Floor
  Cast To Double5 : DataTypeConversion  OutDataTypeStr=double  SaturateOnIntegerOverflow=off  RndMeth=Floor
  Constant1 : Constant  Value=-1
  Constant2 : Constant  Value=-1
  Constant3 : Constant  Value=-1
  Constant4 : Constant  Value=0.5
  Demux2 : Demux  Outputs=3
  Demux3 : Demux  Outputs=3
  Divide : Product  Inputs=*/
  Divide1 : Product  Inputs=*/
  Divide2 : Product  Inputs=*/
  From7 : From  Commented=on  GotoTag=v_a_norm
  From8 : From  Commented=on  GotoTag=q_a
  From9 : From  Commented=on  GotoTag=carrier
  Gain : Gain  Gain=-1/2
  Gain{3..8} (6 alike) : Gain  Gain=G_pulse
  Goto : Goto  Commented=on  GotoTag=v_a_norm
  Goto2 : Goto  Commented=on  GotoTag=q_a
  Goto3 : Goto  Commented=on  GotoTag=carrier
  Max : MinMax  Function=max  Inputs=3
  Max1 : MinMax  Inputs=3
  Mux : Mux  Inputs=6
  Relational Operator : RelationalOperator  OutDataTypeStr=boolean  RndMeth=Simplest  InputSameDT=off
  Relational Operator1 : RelationalOperator  OutDataTypeStr=boolean  RndMeth=Simplest  InputSameDT=off
  Relational Operator2 : RelationalOperator  OutDataTypeStr=boolean  RndMeth=Simplest  InputSameDT=off
  Saturation : Saturate  UpperLimit=1  LowerLimit=0
  Saturation1 : Saturate  UpperLimit=1  LowerLimit=0
  Saturation2 : Saturate  UpperLimit=1  LowerLimit=0
  Scope : Scope  Commented=on  NumInputPorts=3
      settings: ActiveDisplayYMinimum=-0.12499999999999997  ActiveDisplayYMaximum=1.125  DataLoggingVariableName=ScopeData4
  Sum3 : Sum  Inputs=+|+
  Sum4 : Sum  Inputs=|++
  Sum5 : Sum  Inputs=|++
  Sum6 : Sum  Inputs=|++
  Gates : Outport
  wires:
  Vdc/1 -> [V_dc]
  Demux2/3 -> Max1/3, Max/3
  Demux2/1 -> Max1/1, Max/1
  Demux2/2 -> Max1/2, Max/2
  Max/1 -> Sum3/1
  Max1/1 -> Sum3/2
  Sum3/1 -> Gain/1
  Demux3/1 -> Add/2
  Demux3/2 -> Add1/2
  Demux3/3 -> Add2/2
  Sum5/1 -> Abs4/1
  Divide/1 -> Add3/1
  [v_a_mod] -> Divide/1  "v_a_mod"
  Constant3/1 -> Sum6/2
  Cast To Double4/1 -> Sum5/1, Gain4/1  "q_b"
  Constant2/1 -> Sum5/2
  Constant1/1 -> Sum4/2
  Cast To Double5/1 -> Sum6/1, Gain5/1  "q_c"
  Constant4/1 -> Add3/2, Add4/2, Add5/2
  Cast To Double3/1 -> Sum4/1, Goto2/1, Gain3/1  "q_a"
  Abs3/1 -> Gain6/1
  Sum4/1 -> Abs3/1
  Add3/1 -> Saturation/1
  Relational Operator/1 -> Cast To Double3/1
  Saturation2/1 -> Relational Operator2/1
  Saturation/1 -> Goto/1, Relational Operator/1
  Abs4/1 -> Gain7/1
  Carrier/1 -> Relational Operator2/2, Relational Operator1/2, Relational Operator/2, Goto3/1
  [V_dc] -> Divide2/2, Divide1/2, Divide/2
  Sum6/1 -> Abs5/1
  Divide1/1 -> Add4/1
  [v_b_mod] -> Divide1/1  "v_b_mod"
  Abs5/1 -> Gain8/1
  Saturation1/1 -> Relational Operator1/1
  Add5/1 -> Saturation2/1
  Relational Operator1/1 -> Cast To Double4/1
  Add4/1 -> Saturation1/1
  Divide2/1 -> Add5/1
  Relational Operator2/1 -> Cast To Double5/1
  Vabc/1 -> [v_abc]
  [v_abc] -> Demux2/1
  [v_abc] -> Demux3/1
  Gain/1 -> [v_cm]
  [v_cm] -> Add2/1, Add1/1, Add/1
  Add/1 -> [v_a_mod]
  Add1/1 -> [v_b_mod]
  Add2/1 -> [v_c_mod]
  [v_c_mod] -> Divide2/1  "v_c_mod"
  From7/1 -> Scope/1
  From8/1 -> Scope/2
  From9/1 -> Scope/3
  Mux/1 -> Gates/1
  Gain8/1 -> Mux/6  "CL"
  Gain6/1 -> Mux/2  "AL"
  Gain3/1 -> Mux/1  "AH"
  Gain4/1 -> Mux/3  "BH"
  Gain7/1 -> Mux/4  "BL"
  Gain5/1 -> Mux/5  "CH"

== matlab function FS_PWT_Full_Assembly/Simple simulation/MATLAB Function4 ==
  data: T_lim_pos output; T_ref input; T_lim_neg output; nm_ref input; nm_saturation output
function [T_lim_pos, T_lim_neg, nm_saturation]  = Compute_T_n_limits(T_ref, nm_ref)

if T_ref >= 0
    T_lim_pos = T_ref;
    T_lim_neg = 0;
    nm_saturation = nm_ref;
    
else
    T_lim_pos = 0;
    T_lim_neg = T_ref;
    nm_saturation = -nm_ref;
end

== matlab function FS_PWT_Full_Assembly/Simple simulation/MATLAB Function ==
  data: time input; T_ref output; T1 input; T2 input; t0 input; t1 input; t2 input
function T_ref  = Reference_simulation(time, T1,T2, t0, t1, t2)

T_ref = 0;

if time > 0 && time <= t0
    T_ref = 0;

elseif time > t0 && time <= t1
    T_ref = T1;

elseif time > t1 && time <= t1+0.1
    T_ref = T1+(T2-T1)/0.1*(time-t1);

elseif time > t1+0.1 && time <= t2
    T_ref = T2;

elseif time > t2
    T_ref = 0;

end

== matlab function FS_PWT_Full_Assembly/Simple simulation/MATLAB Function2 ==
  data: TL output; n_m input
function TL  = Load_simulation(n_m)

w_m = n_m*pi/30;
K_l = 1*10^(-5)*pi/30;
K_q = 2*10^(-5)*pi/30;
K0 = 1;
TL = 0;

if w_m < 300*pi/30
    TL = 0;
else
    TL = K0 + K_l*w_m + K_q*w_m^2;

end

== matlab function FS_PWT_Full_Assembly/Real log simulation/MATLAB Function1 ==
  data: TL output; n_m input
function TL  = Load_simulation(n_m)

w_m = n_m*pi/30;
K_l = 1*10^(-5)*pi/30;
K_q = 2*10^(-5)*pi/30;
K0 = 1;
TL = 0;

if w_m < 300*pi/30
    TL = 0;
else
    TL = K0 + K_l*w_m + K_q*w_m^2;

end

== matlab function FS_PWT_Full_Assembly/Real log simulation/MATLAB Function3 ==
  data: t_sim input; T_ref output; matrice input
function T_ref = input_from_log(t_sim, matrice)
% Ingressi:
%   t_sim   : tempo corrente della simulazione Simulink (scalare >= 0)
%   matrice : matrice Nx2 [tempo_tabella, coppia_tabella]
% Output:
%   T_ref   : coppia di riferimento interpolata linearmente

    % Vettori temporali e di coppia estratti dalla matrice
    t_data = matrice(:, 1);
    T_data = matrice(:, 2);
    
    % Traslazione del tempo: quando t_sim = 0, t_target corrisponde a t_data(1)
    t_target = t_sim + t_data(1);
    
    % Gestione dei limiti temporali (saturazione agli estremi)
    if t_target <= t_data(1)
        T_ref = T_data(1);
    elseif t_target >= t_data(end)
        T_ref = T_data(end);
    else
        % Ricerca dell'intervallo k tale che: t_data(k) <= t_target < t_data(k+1)
        idx = 1;
        for k = 1:length(t_data)-1
            if t_target >= t_data(k) && t_target <= t_data(k+1)
                idx = k;
                break;
            end
        end
        
        % Coordinate dei due estremi del segmento
        t0 = t_data(idx);
        t1 = t_data(idx+1);
        y0 = T_data(idx);
        y1 = T_data(idx+1);
        
        % Formula dell'interpolazione lineare
        dt = t1 - t0;
        if dt > 0
            alpha = (t_target - t0) / dt;
            T_ref = y0 + alpha * (y1 - y0);
        else
            T_ref = y0; % Protezione contro eventuali istanti coincidenti consecutivi
        end
    end
end

== matlab function FS_PWT_Full_Assembly/Real log simulation/MATLAB Function4 ==
  data: T_lim_pos output; T_ref input; T_lim_neg output; nm_ref input; nm_saturation output
function [T_lim_pos, T_lim_neg, nm_saturation]  = Compute_T_n_limits(T_ref, nm_ref)

if T_ref >= 0
    T_lim_pos = T_ref;
    T_lim_neg = 0;
    nm_saturation = nm_ref;
    
else
    T_lim_pos = 0;
    T_lim_neg = T_ref;
    nm_saturation = -nm_ref;
end
